simulink model "Main_SpeedOptimisedVersionTannenweg"  (R2024b)
settings: Solver=ode15s  StartTime=0.0  StopTime=3600*2  FixedStep=0.1  RelTol=0.001
model workspace (MAT data in the model file):
  Ti = 5
  fa = 0.00071
  fd = 0.03
  ips = 36
  ma = 0.0013
  md = 0.04
  roomarea1 = 20
  s = 15
libraries: fl_lib x1434, nesl_utility x105, SimscapeFluids_lib x35
(part 7 of 22)

== system Main_SpeedOptimisedVersionTannenweg/OG1/Pipe to 11 ==
  Perfect Insulator3 : fl_lib/Thermal/Thermal Elements/Perfect Insulator  T_specify=off  T_priority=None  T=293.15 K  T_nominal_specify=off  T_nominal_value=1  T_nominal_unit=K
  Pipe (TL)3 : fl_lib/Thermal Liquid/Elements/Pipe (TL)  length=5.32 m  area=fa m^2  Dh=fd m  length_add=1 m  roughness=15e-6 m  Re_lam=2000  Re_tur=4000  shape_factor=64  Nu_lam=3.66  dynamic_compressibility=true  inertia=false  p0=0.101325 MPa  T0=293.15 K  mdot0=0 kg/s
  out : PMIOPort  Side=Right
  in : PMIOPort  Port=2  Side=Left
  connections:
  Perfect Insulator3/LConn1 -- Pipe (TL)3/LConn2
  in/RConn1 -- Pipe (TL)3/LConn1
  out/RConn1 -- Pipe (TL)3/RConn1

== system Main_SpeedOptimisedVersionTannenweg/OG1/Pipe to 12 ==
  Perfect Insulator3 : fl_lib/Thermal/Thermal Elements/Perfect Insulator  T_specify=off  T_priority=None  T=293.15 K  T_nominal_specify=off  T_nominal_value=1  T_nominal_unit=K
  Pipe (TL)3 : fl_lib/Thermal Liquid/Elements/Pipe (TL)  length=7.7 m  area=fa m^2  Dh=fd m  length_add=1 m  roughness=15e-6 m  Re_lam=2000  Re_tur=4000  shape_factor=64  Nu_lam=3.66  dynamic_compressibility=true  inertia=false  p0=0.101325 MPa  T0=293.15 K  mdot0=0 kg/s
  out : PMIOPort  Side=Right
  in : PMIOPort  Port=2  Side=Left
  connections:
  in/RConn1 -- Pipe (TL)3/LConn1
  Perfect Insulator3/LConn1 -- Pipe (TL)3/LConn2
  out/RConn1 -- Pipe (TL)3/RConn1

== system Main_SpeedOptimisedVersionTannenweg/OG1/Pipe to 2 ==
  Perfect Insulator1 : fl_lib/Thermal/Thermal Elements/Perfect Insulator  T_specify=off  T_priority=None  T=293.15 K  T_nominal_specify=off  T_nominal_value=1  T_nominal_unit=K
  Pipe (TL)1 : fl_lib/Thermal Liquid/Elements/Pipe (TL)  length=2.38 m  area=fa m^2  Dh=fd m  length_add=1 m  roughness=15e-6 m  Re_lam=2000  Re_tur=4000  shape_factor=64  Nu_lam=3.66  dynamic_compressibility=true  inertia=false  p0=0.101325 MPa  T0=293.15 K  mdot0=0 kg/s
  " in" : PMIOPort  Side=Left
  out : PMIOPort  Port=2  Side=Right
  connections:
  " in"/RConn1 -- Pipe (TL)1/LConn1
  Perfect Insulator1/LConn1 -- Pipe (TL)1/LConn2
  out/RConn1 -- Pipe (TL)1/RConn1

== system Main_SpeedOptimisedVersionTannenweg/OG1/Pipe to 4 ==
  Perfect Insulator2 : fl_lib/Thermal/Thermal Elements/Perfect Insulator  T_specify=off  T_priority=None  T=293.15 K  T_nominal_specify=off  T_nominal_value=1  T_nominal_unit=K
  Pipe (TL)2 : fl_lib/Thermal Liquid/Elements/Pipe (TL)  length=7.38 m  area=fa m^2  Dh=fd m  length_add=1 m  roughness=15e-6 m  Re_lam=2000  Re_tur=4000  shape_factor=64  Nu_lam=3.66  dynamic_compressibility=true  inertia=false  p0=0.101325 MPa  T0=293.15 K  mdot0=0 kg/s
  in : PMIOPort  Side=Left
  out : PMIOPort  Port=2  Side=Right
  connections:
  Pipe (TL)2/LConn1 -- in/RConn1
  Perfect Insulator2/LConn1 -- Pipe (TL)2/LConn2
  out/RConn1 -- Pipe (TL)2/RConn1

== system Main_SpeedOptimisedVersionTannenweg/OG1/Pipe to 5 ==
  Perfect Insulator3 : fl_lib/Thermal/Thermal Elements/Perfect Insulator  T_specify=off  T_priority=None  T=293.15 K  T_nominal_specify=off  T_nominal_value=1  T_nominal_unit=K
  Pipe (TL)3 : fl_lib/Thermal Liquid/Elements/Pipe (TL)  length=12.42 m  area=fa m^2  Dh=fd m  length_add=1 m  roughness=15e-6 m  Re_lam=2000  Re_tur=4000  shape_factor=64  Nu_lam=3.66  dynamic_compressibility=true  inertia=false  p0=0.101325 MPa  T0=293.15 K  mdot0=0 kg/s
  out : PMIOPort  Side=Right
  " in" : PMIOPort  Port=2  Side=Left
  connections:
  " in"/RConn1 -- Pipe (TL)3/LConn1
  Perfect Insulator3/LConn1 -- Pipe (TL)3/LConn2
  out/RConn1 -- Pipe (TL)3/RConn1

== system Main_SpeedOptimisedVersionTannenweg/OG1/Pipe to 6 ==
  Perfect Insulator3 : fl_lib/Thermal/Thermal Elements/Perfect Insulator  T_specify=off  T_priority=None  T=293.15 K  T_nominal_specify=off  T_nominal_value=1  T_nominal_unit=K
  Pipe (TL)3 : fl_lib/Thermal Liquid/Elements/Pipe (TL)  length=9.34 m  area=fa m^2  Dh=fd m  length_add=1 m  roughness=15e-6 m  Re_lam=2000  Re_tur=4000  shape_factor=64  Nu_lam=3.66  dynamic_compressibility=true  inertia=false  p0=0.101325 MPa  T0=293.15 K  mdot0=0 kg/s
  out : PMIOPort  Side=Right
  " in" : PMIOPort  Port=2  Side=Left
  connections:
  Perfect Insulator3/LConn1 -- Pipe (TL)3/LConn2
  " in"/RConn1 -- Pipe (TL)3/LConn1
  out/RConn1 -- Pipe (TL)3/RConn1

== system Main_SpeedOptimisedVersionTannenweg/OG1/Pipe to 7 ==
  Perfect Insulator3 : fl_lib/Thermal/Thermal Elements/Perfect Insulator  T_specify=off  T_priority=None  T=293.15 K  T_nominal_specify=off  T_nominal_value=1  T_nominal_unit=K
  Pipe (TL)3 : fl_lib/Thermal Liquid/Elements/Pipe (TL)  length=3.5 m  area=fa m^2  Dh=fd m  length_add=1 m  roughness=15e-6 m  Re_lam=2000  Re_tur=4000  shape_factor=64  Nu_lam=3.66  dynamic_compressibility=true  inertia=false  p0=0.101325 MPa  T0=293.15 K  mdot0=0 kg/s
  out : PMIOPort  Side=Right
  " in" : PMIOPort  Port=2  Side=Left
  connections:
  " in"/RConn1 -- Pipe (TL)3/LConn1
  Perfect Insulator3/LConn1 -- Pipe (TL)3/LConn2
  out/RConn1 -- Pipe (TL)3/RConn1

== system Main_SpeedOptimisedVersionTannenweg/OG1/Pipe to 8 ==
  Perfect Insulator3 : fl_lib/Thermal/Thermal Elements/Perfect Insulator  T_specify=off  T_priority=None  T=293.15 K  T_nominal_specify=off  T_nominal_value=1  T_nominal_unit=K
  Pipe (TL)3 : fl_lib/Thermal Liquid/Elements/Pipe (TL)  length=10.04 m  area=fa m^2  Dh=fd m  length_add=1 m  roughness=15e-6 m  Re_lam=2000  Re_tur=4000  shape_factor=64  Nu_lam=3.66  dynamic_compressibility=true  inertia=false  p0=0.101325 MPa  T0=293.15 K  mdot0=0 kg/s
  out : PMIOPort  Side=Right
  in : PMIOPort  Port=2  Side=Left
  connections:
  in/RConn1 -- Pipe (TL)3/LConn1
  Perfect Insulator3/LConn1 -- Pipe (TL)3/LConn2
  out/RConn1 -- Pipe (TL)3/RConn1

== system Main_SpeedOptimisedVersionTannenweg/OG1/Pipe to 9a ==
  Perfect Insulator3 : fl_lib/Thermal/Thermal Elements/Perfect Insulator  T_specify=off  T_priority=None  T=293.15 K  T_nominal_specify=off  T_nominal_value=1  T_nominal_unit=K
  Pipe (TL)3 : fl_lib/Thermal Liquid/Elements/Pipe (TL)  length=10.14 m  area=fa m^2  Dh=fd m  length_add=1 m  roughness=15e-6 m  Re_lam=2000  Re_tur=4000  shape_factor=64  Nu_lam=3.66  dynamic_compressibility=true  inertia=false  p0=0.101325 MPa  T0=293.15 K  mdot0=0 kg/s
  out : PMIOPort  Side=Right
  in : PMIOPort  Port=2  Side=Left
  connections:
  Perfect Insulator3/LConn1 -- Pipe (TL)3/LConn2
  in/RConn1 -- Pipe (TL)3/LConn1
  Pipe (TL)3/RConn1 -- out/RConn1

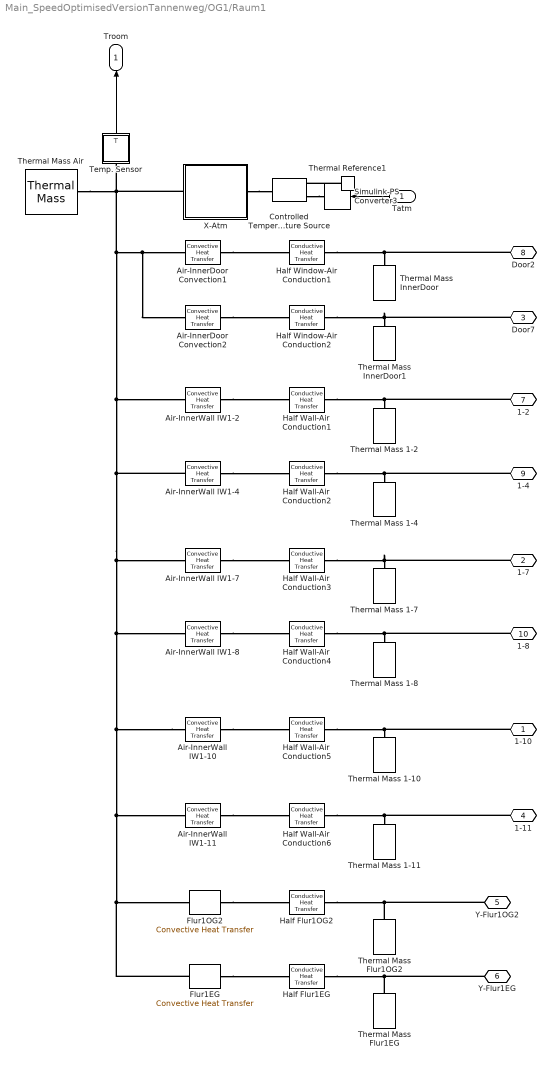
== system Main_SpeedOptimisedVersionTannenweg/OG1/Raum1 ==
  Tatm : Inport
  Air-InnerDoor Convection1 : fl_lib/Thermal/Thermal Elements/Convective Heat Transfer  thermal_type=foundation.enum.constant_variable.constant  area=2 m^2  heat_tr_coeff=.8 W/m^2/K  min_heat_tr_coeff=1e-3 W/(K*m^2)  T_specify=off  T_priority=High  T=0 K  T_nominal_specify=off  T_nominal_value=1  T_nominal_unit=K  Q_specify=off  Q_priority=High  Q=0 J/s  Q_nominal_specify=off  Q_nominal_value=1  Q_nominal_unit=W
  Air-InnerDoor Convection2 : fl_lib/Thermal/Thermal Elements/Convective Heat Transfer  thermal_type=foundation.enum.constant_variable.constant  area=2 m^2  heat_tr_coeff=.8 W/m^2/K  min_heat_tr_coeff=1e-3 W/(K*m^2)  T_specify=off  T_priority=High  T=0 K  T_nominal_specify=off  T_nominal_value=1  T_nominal_unit=K  Q_specify=off  Q_priority=High  Q=0 J/s  Q_nominal_specify=off  Q_nominal_value=1  Q_nominal_unit=W
  Air-InnerWall IW1-10 : fl_lib/Thermal/Thermal Elements/Convective Heat Transfer  thermal_type=foundation.enum.constant_variable.constant  area=3.5 m^2  heat_tr_coeff=.8 W/m^2/K  min_heat_tr_coeff=1e-3 W/(K*m^2)  T_specify=off  T_priority=High  T=0 K  T_nominal_specify=off  T_nominal_value=1  T_nominal_unit=K  Q_specify=off  Q_priority=High  Q=0 J/s  Q_nominal_specify=off  Q_nominal_value=1  Q_nominal_unit=W
  Air-InnerWall IW1-11 : fl_lib/Thermal/Thermal Elements/Convective Heat Transfer  thermal_type=foundation.enum.constant_variable.constant  area=3.7 m^2  heat_tr_coeff=.8 W/m^2/K  min_heat_tr_coeff=1e-3 W/(K*m^2)  T_specify=off  T_priority=High  T=0 K  T_nominal_specify=off  T_nominal_value=1  T_nominal_unit=K  Q_specify=off  Q_priority=High  Q=0 J/s  Q_nominal_specify=off  Q_nominal_value=1  Q_nominal_unit=W
  Air-InnerWall IW1-2 : fl_lib/Thermal/Thermal Elements/Convective Heat Transfer  thermal_type=foundation.enum.constant_variable.constant  area=3.8 m^2  heat_tr_coeff=.8 W/m^2/K  min_heat_tr_coeff=1e-3 W/(K*m^2)  T_specify=off  T_priority=High  T=0 K  T_nominal_specify=off  T_nominal_value=1  T_nominal_unit=K  Q_specify=off  Q_priority=High  Q=0 J/s  Q_nominal_specify=off  Q_nominal_value=1  Q_nominal_unit=W
  Air-InnerWall IW1-4 : fl_lib/Thermal/Thermal Elements/Convective Heat Transfer  thermal_type=foundation.enum.constant_variable.constant  area=7.2 m^2  heat_tr_coeff=.8 W/m^2/K  min_heat_tr_coeff=1e-3 W/(K*m^2)  T_specify=off  T_priority=High  T=0 K  T_nominal_specify=off  T_nominal_value=1  T_nominal_unit=K  Q_specify=off  Q_priority=High  Q=0 J/s  Q_nominal_specify=off  Q_nominal_value=1  Q_nominal_unit=W
  Air-InnerWall IW1-7 : fl_lib/Thermal/Thermal Elements/Convective Heat Transfer  thermal_type=foundation.enum.constant_variable.constant  area=3.1 m^2  heat_tr_coeff=.8 W/m^2/K  min_heat_tr_coeff=1e-3 W/(K*m^2)  T_specify=off  T_priority=High  T=0 K  T_nominal_specify=off  T_nominal_value=1  T_nominal_unit=K  Q_specify=off  Q_priority=High  Q=0 J/s  Q_nominal_specify=off  Q_nominal_value=1  Q_nominal_unit=W
  Air-InnerWall IW1-8 : fl_lib/Thermal/Thermal Elements/Convective Heat Transfer  thermal_type=foundation.enum.constant_variable.constant  area=7.9 m^2  heat_tr_coeff=.8 W/m^2/K  min_heat_tr_coeff=1e-3 W/(K*m^2)  T_specify=off  T_priority=High  T=0 K  T_nominal_specify=off  T_nominal_value=1  T_nominal_unit=K  Q_specify=off  Q_priority=High  Q=0 J/s  Q_nominal_specify=off  Q_nominal_value=1  Q_nominal_unit=W
  Controlled Temperature Source : fl_lib/Thermal/Thermal Sources/Controlled Temperature Source
  Flur1EG : fl_lib/Thermal/Thermal Elements/Convective Heat Transfer  thermal_type=foundation.enum.constant_variable.constant  area=10.76 m^2  heat_tr_coeff=.8 W/m^2/K  min_heat_tr_coeff=1e-3 W/(K*m^2)  T_specify=off  T_priority=High  T=0 K  T_nominal_specify=off  T_nominal_value=1  T_nominal_unit=K  Q_specify=off  Q_priority=High  Q=0 J/s  Q_nominal_specify=off  Q_nominal_value=1  Q_nominal_unit=W
  Flur1OG2 : fl_lib/Thermal/Thermal Elements/Convective Heat Transfer  thermal_type=foundation.enum.constant_variable.constant  area=10.76 m^2  heat_tr_coeff=.8 W/m^2/K  min_heat_tr_coeff=1e-3 W/(K*m^2)  T_specify=off  T_priority=High  T=0 K  T_nominal_specify=off  T_nominal_value=1  T_nominal_unit=K  Q_specify=off  Q_priority=High  Q=0 J/s  Q_nominal_specify=off  Q_nominal_value=1  Q_nominal_unit=W
  Half Flur1EG : fl_lib/Thermal/Thermal Elements/Conductive Heat Transfer  thermal_type=foundation.enum.ConstantVariableTabulated.Constant  wall_geometry=foundation.enum.ConductionWallGeometry.Planar  area=10.76 m^2  thickness=.15 m  d_in=0.05 m  d_out=0.1 m  L=1 m  th_cond_min=10 W/(K*m)  th_cond=.32 W/m/K  th_cond_TLU=[413, 401, 392, 383, 371, 357, 342] W/(K*m)  temp_TLU=[200, 273, 400, 600, 800, 1000, 1200] K  T_specify=off  T_priority=High  T=0 K  T_nominal_specify=off  T_nominal_value=1  T_nominal_unit=K  Q_specify=off  Q_priority=High  Q=0 J/s  Q_nominal_specify=off  Q_nominal_value=1  Q_nominal_unit=W
  Half Flur1OG2 : fl_lib/Thermal/Thermal Elements/Conductive Heat Transfer  thermal_type=foundation.enum.ConstantVariableTabulated.Constant  wall_geometry=foundation.enum.ConductionWallGeometry.Planar  area=10.76 m^2  thickness=.15 m  d_in=0.05 m  d_out=0.1 m  L=1 m  th_cond_min=10 W/(K*m)  th_cond=.32 W/m/K  th_cond_TLU=[413, 401, 392, 383, 371, 357, 342] W/(K*m)  temp_TLU=[200, 273, 400, 600, 800, 1000, 1200] K  T_specify=off  T_priority=High  T=0 K  T_nominal_specify=off  T_nominal_value=1  T_nominal_unit=K  Q_specify=off  Q_priority=High  Q=0 J/s  Q_nominal_specify=off  Q_nominal_value=1  Q_nominal_unit=W
  Half Wall-Air Conduction1 : fl_lib/Thermal/Thermal Elements/Conductive Heat Transfer  thermal_type=foundation.enum.ConstantVariableTabulated.Constant  wall_geometry=foundation.enum.ConductionWallGeometry.Planar  area=3.8 m^2  thickness=.16 m  d_in=0.05 m  d_out=0.1 m  L=1 m  th_cond_min=10 W/(K*m)  th_cond=.069 W/m/K  th_cond_TLU=[413, 401, 392, 383, 371, 357, 342] W/(K*m)  temp_TLU=[200, 273, 400, 600, 800, 1000, 1200] K  T_specify=off  T_priority=High  T=0 K  T_nominal_specify=off  T_nominal_value=1  T_nominal_unit=K  Q_specify=off  Q_priority=High  Q=0 J/s  Q_nominal_specify=off  Q_nominal_value=1  Q_nominal_unit=W
  Half Wall-Air Conduction2 : fl_lib/Thermal/Thermal Elements/Conductive Heat Transfer  thermal_type=foundation.enum.ConstantVariableTabulated.Constant  wall_geometry=foundation.enum.ConductionWallGeometry.Planar  area=7.2 m^2  thickness=.16 m  d_in=0.05 m  d_out=0.1 m  L=1 m  th_cond_min=10 W/(K*m)  th_cond=.069 W/m/K  th_cond_TLU=[413, 401, 392, 383, 371, 357, 342] W/(K*m)  temp_TLU=[200, 273, 400, 600, 800, 1000, 1200] K  T_specify=off  T_priority=High  T=0 K  T_nominal_specify=off  T_nominal_value=1  T_nominal_unit=K  Q_specify=off  Q_priority=High  Q=0 J/s  Q_nominal_specify=off  Q_nominal_value=1  Q_nominal_unit=W
  Half Wall-Air Conduction3 : fl_lib/Thermal/Thermal Elements/Conductive Heat Transfer  thermal_type=foundation.enum.ConstantVariableTabulated.Constant  wall_geometry=foundation.enum.ConductionWallGeometry.Planar  area=3.1 m^2  thickness=.16 m  d_in=0.05 m  d_out=0.1 m  L=1 m  th_cond_min=10 W/(K*m)  th_cond=.069 W/m/K  th_cond_TLU=[413, 401, 392, 383, 371, 357, 342] W/(K*m)  temp_TLU=[200, 273, 400, 600, 800, 1000, 1200] K  T_specify=off  T_priority=High  T=0 K  T_nominal_specify=off  T_nominal_value=1  T_nominal_unit=K  Q_specify=off  Q_priority=High  Q=0 J/s  Q_nominal_specify=off  Q_nominal_value=1  Q_nominal_unit=W
  Half Wall-Air Conduction4 : fl_lib/Thermal/Thermal Elements/Conductive Heat Transfer  thermal_type=foundation.enum.ConstantVariableTabulated.Constant  wall_geometry=foundation.enum.ConductionWallGeometry.Planar  area=7.9 m^2  thickness=.16 m  d_in=0.05 m  d_out=0.1 m  L=1 m  th_cond_min=10 W/(K*m)  th_cond=.069 W/m/K  th_cond_TLU=[413, 401, 392, 383, 371, 357, 342] W/(K*m)  temp_TLU=[200, 273, 400, 600, 800, 1000, 1200] K  T_specify=off  T_priority=High  T=0 K  T_nominal_specify=off  T_nominal_value=1  T_nominal_unit=K  Q_specify=off  Q_priority=High  Q=0 J/s  Q_nominal_specify=off  Q_nominal_value=1  Q_nominal_unit=W
  Half Wall-Air Conduction5 : fl_lib/Thermal/Thermal Elements/Conductive Heat Transfer  thermal_type=foundation.enum.ConstantVariableTabulated.Constant  wall_geometry=foundation.enum.ConductionWallGeometry.Planar  area=3.5 m^2  thickness=.16 m  d_in=0.05 m  d_out=0.1 m  L=1 m  th_cond_min=10 W/(K*m)  th_cond=.069 W/m/K  th_cond_TLU=[413, 401, 392, 383, 371, 357, 342] W/(K*m)  temp_TLU=[200, 273, 400, 600, 800, 1000, 1200] K  T_specify=off  T_priority=High  T=0 K  T_nominal_specify=off  T_nominal_value=1  T_nominal_unit=K  Q_specify=off  Q_priority=High  Q=0 J/s  Q_nominal_specify=off  Q_nominal_value=1  Q_nominal_unit=W
  Half Wall-Air Conduction6 : fl_lib/Thermal/Thermal Elements/Conductive Heat Transfer  thermal_type=foundation.enum.ConstantVariableTabulated.Constant  wall_geometry=foundation.enum.ConductionWallGeometry.Planar  area=3.7 m^2  thickness=.16 m  d_in=0.05 m  d_out=0.1 m  L=1 m  th_cond_min=10 W/(K*m)  th_cond=.069 W/m/K  th_cond_TLU=[413, 401, 392, 383, 371, 357, 342] W/(K*m)  temp_TLU=[200, 273, 400, 600, 800, 1000, 1200] K  T_specify=off  T_priority=High  T=0 K  T_nominal_specify=off  T_nominal_value=1  T_nominal_unit=K  Q_specify=off  Q_priority=High  Q=0 J/s  Q_nominal_specify=off  Q_nominal_value=1  Q_nominal_unit=W
  Half Window-Air Conduction1 : fl_lib/Thermal/Thermal Elements/Conductive Heat Transfer  thermal_type=foundation.enum.ConstantVariableTabulated.Constant  wall_geometry=foundation.enum.ConductionWallGeometry.Planar  area=2 m^2  thickness=.022 m  d_in=0.05 m  d_out=0.1 m  L=1 m  th_cond_min=10 W/(K*m)  th_cond=.13 W/m/K  th_cond_TLU=[413, 401, 392, 383, 371, 357, 342] W/(K*m)  temp_TLU=[200, 273, 400, 600, 800, 1000, 1200] K  T_specify=off  T_priority=High  T=0 K  T_nominal_specify=off  T_nominal_value=1  T_nominal_unit=K  Q_specify=off  Q_priority=High  Q=0 J/s  Q_nominal_specify=off  Q_nominal_value=1  Q_nominal_unit=W
  Half Window-Air Conduction2 : fl_lib/Thermal/Thermal Elements/Conductive Heat Transfer  thermal_type=foundation.enum.ConstantVariableTabulated.Constant  wall_geometry=foundation.enum.ConductionWallGeometry.Planar  area=2 m^2  thickness=.022 m  d_in=0.05 m  d_out=0.1 m  L=1 m  th_cond_min=10 W/(K*m)  th_cond=.13 W/m/K  th_cond_TLU=[413, 401, 392, 383, 371, 357, 342] W/(K*m)  temp_TLU=[200, 273, 400, 600, 800, 1000, 1200] K  T_specify=off  T_priority=High  T=0 K  T_nominal_specify=off  T_nominal_value=1  T_nominal_unit=K  Q_specify=off  Q_priority=High  Q=0 J/s  Q_nominal_specify=off  Q_nominal_value=1  Q_nominal_unit=W
  Simulink-PS Converter3 : nesl_utility/Simulink-PS Converter  PhysicalDomain=network_engine_domain  SubClassName=ps_input  LeftPortType=input  RightPortType=output  PseudoPeriodic=off  Frequencies=[]  NoiseDistribution=none  NoiseParameters=[]  Unit=degC  AffineConversion=on  FilteringAndDerivatives=zero  SimscapeFilterOrder=1  InputFilterTimeConstant=.001  UdotUserProvided=0
  Temp. Sensor : Subsystem
  Thermal Mass 1-10 : fl_lib/Thermal/Thermal Elements/Thermal Mass  mass_type=foundation.enum.constant_variable.constant  mass=3.5*.15*547 kg  sp_heat=876 J/kg/K  mass_min=1e-6 kg  num_ports=foundation.enum.numPorts2.one  m_specify=off  m_priority=High  m=1 kg  m_nominal_specify=off  m_nominal_value=1  m_nominal_unit=kg  T_specify=on  T_priority=High  T=Ti degC  T_nominal_specify=off  T_nominal_value=1  T_nominal_unit=K  Q_specify=off  Q_priority=None  Q=0 W  Q_nominal_specify=off  Q_nominal_value=1  Q_nominal_unit=W
  Thermal Mass 1-11 : fl_lib/Thermal/Thermal Elements/Thermal Mass  mass_type=foundation.enum.constant_variable.constant  mass=3.7*.15*547 kg  sp_heat=876 J/kg/K  mass_min=1e-6 kg  num_ports=foundation.enum.numPorts2.one  m_specify=off  m_priority=High  m=1 kg  m_nominal_specify=off  m_nominal_value=1  m_nominal_unit=kg  T_specify=on  T_priority=High  T=Ti degC  T_nominal_specify=off  T_nominal_value=1  T_nominal_unit=K  Q_specify=off  Q_priority=None  Q=0 W  Q_nominal_specify=off  Q_nominal_value=1  Q_nominal_unit=W
  Thermal Mass 1-2 : fl_lib/Thermal/Thermal Elements/Thermal Mass  mass_type=foundation.enum.constant_variable.constant  mass=3.8*.15*547 kg  sp_heat=876 J/kg/K  mass_min=1e-6 kg  num_ports=foundation.enum.numPorts2.one  m_specify=off  m_priority=High  m=1 kg  m_nominal_specify=off  m_nominal_value=1  m_nominal_unit=kg  T_specify=on  T_priority=High  T=Ti degC  T_nominal_specify=off  T_nominal_value=1  T_nominal_unit=K  Q_specify=off  Q_priority=None  Q=0 W  Q_nominal_specify=off  Q_nominal_value=1  Q_nominal_unit=W
  Thermal Mass 1-4 : fl_lib/Thermal/Thermal Elements/Thermal Mass  mass_type=foundation.enum.constant_variable.constant  mass=7.2*.15*547 kg  sp_heat=876 J/kg/K  mass_min=1e-6 kg  num_ports=foundation.enum.numPorts2.one  m_specify=off  m_priority=High  m=1 kg  m_nominal_specify=off  m_nominal_value=1  m_nominal_unit=kg  T_specify=on  T_priority=High  T=Ti degC  T_nominal_specify=off  T_nominal_value=1  T_nominal_unit=K  Q_specify=off  Q_priority=None  Q=0 W  Q_nominal_specify=off  Q_nominal_value=1  Q_nominal_unit=W
  Thermal Mass 1-7 : fl_lib/Thermal/Thermal Elements/Thermal Mass  mass_type=foundation.enum.constant_variable.constant  mass=3.1*.15*547 kg  sp_heat=876 J/kg/K  mass_min=1e-6 kg  num_ports=foundation.enum.numPorts2.one  m_specify=off  m_priority=High  m=1 kg  m_nominal_specify=off  m_nominal_value=1  m_nominal_unit=kg  T_specify=on  T_priority=High  T=Ti degC  T_nominal_specify=off  T_nominal_value=1  T_nominal_unit=K  Q_specify=off  Q_priority=None  Q=0 W  Q_nominal_specify=off  Q_nominal_value=1  Q_nominal_unit=W
  Thermal Mass 1-8 : fl_lib/Thermal/Thermal Elements/Thermal Mass  mass_type=foundation.enum.constant_variable.constant  mass=7.9*.15*547 kg  sp_heat=876 J/kg/K  mass_min=1e-6 kg  num_ports=foundation.enum.numPorts2.one  m_specify=off  m_priority=High  m=1 kg  m_nominal_specify=off  m_nominal_value=1  m_nominal_unit=kg  T_specify=on  T_priority=High  T=Ti degC  T_nominal_specify=off  T_nominal_value=1  T_nominal_unit=K  Q_specify=off  Q_priority=None  Q=0 W  Q_nominal_specify=off  Q_nominal_value=1  Q_nominal_unit=W
  Thermal Mass Air : fl_lib/Thermal/Thermal Elements/Thermal Mass  mass_type=foundation.enum.constant_variable.constant  mass=13.9 kg  sp_heat=1005 J/kg/K  mass_min=1e-6 kg  num_ports=foundation.enum.numPorts2.one  m_specify=off  m_priority=High  m=1 kg  m_nominal_specify=off  m_nominal_value=1  m_nominal_unit=kg  T_specify=on  T_priority=High  T=Ti degC  T_nominal_specify=off  T_nominal_value=1  T_nominal_unit=K  Q_specify=off  Q_priority=None  Q=0 W  Q_nominal_specify=off  Q_nominal_value=1  Q_nominal_unit=W
  Thermal Mass Flur1EG : fl_lib/Thermal/Thermal Elements/Thermal Mass  mass_type=foundation.enum.constant_variable.constant  mass=3033 kg  sp_heat=889 J/kg/K  mass_min=1e-6 kg  num_ports=foundation.enum.numPorts2.one  m_specify=off  m_priority=High  m=1 kg  m_nominal_specify=off  m_nominal_value=1  m_nominal_unit=kg  T_specify=on  T_priority=High  T=Ti degC  T_nominal_specify=off  T_nominal_value=1  T_nominal_unit=K  Q_specify=off  Q_priority=None  Q=0 W  Q_nominal_specify=off  Q_nominal_value=1  Q_nominal_unit=W
  Thermal Mass Flur1OG2 : fl_lib/Thermal/Thermal Elements/Thermal Mass  mass_type=foundation.enum.constant_variable.constant  mass=3033 kg  sp_heat=889 J/kg/K  mass_min=1e-6 kg  num_ports=foundation.enum.numPorts2.one  m_specify=off  m_priority=High  m=1 kg  m_nominal_specify=off  m_nominal_value=1  m_nominal_unit=kg  T_specify=on  T_priority=High  T=Ti degC  T_nominal_specify=off  T_nominal_value=1  T_nominal_unit=K  Q_specify=off  Q_priority=None  Q=0 W  Q_nominal_specify=off  Q_nominal_value=1  Q_nominal_unit=W
  Thermal Mass InnerDoor : fl_lib/Thermal/Thermal Elements/Thermal Mass  mass_type=foundation.enum.constant_variable.constant  mass=2*.022*450 kg  sp_heat=1600 J/kg/K  mass_min=1e-6 kg  num_ports=foundation.enum.numPorts2.one  m_specify=off  m_priority=High  m=1 kg  m_nominal_specify=off  m_nominal_value=1  m_nominal_unit=kg  T_specify=on  T_priority=High  T=Ti degC  T_nominal_specify=off  T_nominal_value=1  T_nominal_unit=K  Q_specify=off  Q_priority=None  Q=0 W  Q_nominal_specify=off  Q_nominal_value=1  Q_nominal_unit=W
  Thermal Mass InnerDoor1 : fl_lib/Thermal/Thermal Elements/Thermal Mass  mass_type=foundation.enum.constant_variable.constant  mass=2*.022*450 kg  sp_heat=1600 J/kg/K  mass_min=1e-6 kg  num_ports=foundation.enum.numPorts2.one  m_specify=off  m_priority=High  m=1 kg  m_nominal_specify=off  m_nominal_value=1  m_nominal_unit=kg  T_specify=on  T_priority=High  T=Ti degC  T_nominal_specify=off  T_nominal_value=1  T_nominal_unit=K  Q_specify=off  Q_priority=None  Q=0 W  Q_nominal_specify=off  Q_nominal_value=1  Q_nominal_unit=W
  Thermal Reference1 : fl_lib/Thermal/Thermal Elements/Thermal Reference
  X-Atm : Subsystem
  1-10 : PMIOPort  Side=Left
  1-7 : PMIOPort  Port=2  Side=Left
  Door7 : PMIOPort  Port=3  Side=Left
  1-11 : PMIOPort  Port=4  Side=Left
  Y-Flur1OG2 : PMIOPort  Port=5  Side=Left
  Y-Flur1EG : PMIOPort  Port=6  Side=Left
  1-2 : PMIOPort  Port=7  Side=Right
  Door2 : PMIOPort  Port=8  Side=Right
  1-4 : PMIOPort  Port=9  Side=Right
  1-8 : PMIOPort  Port=10  Side=Right
  Troom : Outport
  wires:
  Temp. Sensor/1(T) -> Troom/1
  Tatm/1 -> Simulink-PS Converter3/1
  connections:
  Flur1OG2/RConn1 -- Half Flur1OG2/LConn1
  Half Flur1OG2/RConn1 -- Y-Flur1OG2/RConn1 -- Thermal Mass Flur1OG2/LConn1
  Air-InnerDoor Convection1/RConn1 -- Half Window-Air Conduction1/LConn1
  Air-InnerWall IW1-11/RConn1 -- Half Wall-Air Conduction6/LConn1
  Air-InnerWall IW1-7/RConn1 -- Half Wall-Air Conduction3/LConn1
  Air-InnerWall IW1-10/RConn1 -- Half Wall-Air Conduction5/LConn1
  Air-InnerDoor Convection2/RConn1 -- Half Window-Air Conduction2/LConn1
  Air-InnerWall IW1-2/RConn1 -- Half Wall-Air Conduction1/LConn1
  Air-InnerWall IW1-4/RConn1 -- Half Wall-Air Conduction2/LConn1
  Air-InnerWall IW1-8/RConn1 -- Half Wall-Air Conduction4/LConn1
  1-10/RConn1 -- Thermal Mass 1-10/LConn1 -- Half Wall-Air Conduction5/RConn1
  Thermal Mass 1-7/LConn1 -- Half Wall-Air Conduction3/RConn1 -- 1-7/RConn1
  Half Wall-Air Conduction6/RConn1 -- Thermal Mass 1-11/LConn1 -- 1-11/RConn1
  Door2/RConn1 -- Thermal Mass InnerDoor/LConn1 -- Half Window-Air Conduction1/RConn1
  Thermal Mass InnerDoor1/LConn1 -- Door7/RConn1 -- Half Window-Air Conduction2/RConn1
  Half Wall-Air Conduction2/RConn1 -- Thermal Mass 1-4/LConn1 -- 1-4/RConn1
  Half Wall-Air Conduction4/RConn1 -- Thermal Mass 1-8/LConn1 -- 1-8/RConn1
  1-2/RConn1 -- Thermal Mass 1-2/LConn1 -- Half Wall-Air Conduction1/RConn1
  Thermal Reference1/LConn1 -- Controlled Temperature Source/RConn2
  Controlled Temperature Source/RConn1 -- Simulink-PS Converter3/RConn1
  Air-InnerWall IW1-10/LConn1 -- Flur1EG/LConn1 -- Flur1OG2/LConn1 -- Air-InnerWall IW1-11/LConn1 -- Thermal Mass Air/LConn1 -- Temp. Sensor/LConn1 -- X-Atm/LConn1 -- Air-InnerDoor Convection1/LConn1 -- Air-InnerDoor Convection2/LConn1 -- Air-InnerWall IW1-2/LConn1 -- Air-InnerWall IW1-4/LConn1 -- Air-InnerWall IW1-7/LConn1 -- Air-InnerWall IW1-8/LConn1
  X-Atm/RConn1 -- Controlled Temperature Source/LConn1
  Half Flur1EG/RConn1 -- Thermal Mass Flur1EG/LConn1 -- Y-Flur1EG/RConn1
  Flur1EG/RConn1 -- Half Flur1EG/LConn1

== system Main_SpeedOptimisedVersionTannenweg/OG1/Raum10 ==
  valve command : Inport
  Tatm : Inport  Port=2
  Air-InnerDoor Convection1 : fl_lib/Thermal/Thermal Elements/Convective Heat Transfer  thermal_type=foundation.enum.constant_variable.constant  area=1.8 m^2  heat_tr_coeff=.8 W/m^2/K  min_heat_tr_coeff=1e-3 W/(K*m^2)  T_specify=off  T_priority=High  T=0 K  T_nominal_specify=off  T_nominal_value=1  T_nominal_unit=K  Q_specify=off  Q_priority=High  Q=0 J/s  Q_nominal_specify=off  Q_nominal_value=1  Q_nominal_unit=W
  Controlled Temperature Source : fl_lib/Thermal/Thermal Sources/Controlled Temperature Source
  Flur10EG : fl_lib/Thermal/Thermal Elements/Convective Heat Transfer  thermal_type=foundation.enum.constant_variable.constant  area=14.51 m^2  heat_tr_coeff=.8 W/m^2/K  min_heat_tr_coeff=1e-3 W/(K*m^2)  T_specify=off  T_priority=High  T=0 K  T_nominal_specify=off  T_nominal_value=1  T_nominal_unit=K  Q_specify=off  Q_priority=High  Q=0 J/s  Q_nominal_specify=off  Q_nominal_value=1  Q_nominal_unit=W
  Flur10OG2 : fl_lib/Thermal/Thermal Elements/Convective Heat Transfer  thermal_type=foundation.enum.constant_variable.constant  area=14.51 m^2  heat_tr_coeff=.8 W/m^2/K  min_heat_tr_coeff=1e-3 W/(K*m^2)  T_specify=off  T_priority=High  T=0 K  T_nominal_specify=off  T_nominal_value=1  T_nominal_unit=K  Q_specify=off  Q_priority=High  Q=0 J/s  Q_nominal_specify=off  Q_nominal_value=1  Q_nominal_unit=W
  Half Flur10EG : fl_lib/Thermal/Thermal Elements/Conductive Heat Transfer  thermal_type=foundation.enum.ConstantVariableTabulated.Constant  wall_geometry=foundation.enum.ConductionWallGeometry.Planar  area=14.51 m^2  thickness=.15 m  d_in=0.05 m  d_out=0.1 m  L=1 m  th_cond_min=10 W/(K*m)  th_cond=.32 W/m/K  th_cond_TLU=[413, 401, 392, 383, 371, 357, 342] W/(K*m)  temp_TLU=[200, 273, 400, 600, 800, 1000, 1200] K  T_specify=off  T_priority=High  T=0 K  T_nominal_specify=off  T_nominal_value=1  T_nominal_unit=K  Q_specify=off  Q_priority=High  Q=0 J/s  Q_nominal_specify=off  Q_nominal_value=1  Q_nominal_unit=W
  Half Flur10OG2 : fl_lib/Thermal/Thermal Elements/Conductive Heat Transfer  thermal_type=foundation.enum.ConstantVariableTabulated.Constant  wall_geometry=foundation.enum.ConductionWallGeometry.Planar  area=14.51 m^2  thickness=.15 m  d_in=0.05 m  d_out=0.1 m  L=1 m  th_cond_min=10 W/(K*m)  th_cond=.32 W/m/K  th_cond_TLU=[413, 401, 392, 383, 371, 357, 342] W/(K*m)  temp_TLU=[200, 273, 400, 600, 800, 1000, 1200] K  T_specify=off  T_priority=High  T=0 K  T_nominal_specify=off  T_nominal_value=1  T_nominal_unit=K  Q_specify=off  Q_priority=High  Q=0 J/s  Q_nominal_specify=off  Q_nominal_value=1  Q_nominal_unit=W
  Half Wall-Air Conduction1 : fl_lib/Thermal/Thermal Elements/Conductive Heat Transfer  thermal_type=foundation.enum.ConstantVariableTabulated.Constant  wall_geometry=foundation.enum.ConductionWallGeometry.Planar  area=3.7 m^2  thickness=.16 m  d_in=0.05 m  d_out=0.1 m  L=1 m  th_cond_min=10 W/(K*m)  th_cond=.069 W/m/K  th_cond_TLU=[413, 401, 392, 383, 371, 357, 342] W/(K*m)  temp_TLU=[200, 273, 400, 600, 800, 1000, 1200] K  T_specify=off  T_priority=High  T=0 K  T_nominal_specify=off  T_nominal_value=1  T_nominal_unit=K  Q_specify=off  Q_priority=High  Q=0 J/s  Q_nominal_specify=off  Q_nominal_value=1  Q_nominal_unit=W
  Half Wall-Air Conduction2 : fl_lib/Thermal/Thermal Elements/Conductive Heat Transfer  thermal_type=foundation.enum.ConstantVariableTabulated.Constant  wall_geometry=foundation.enum.ConductionWallGeometry.Planar  area=1.8 m^2  thickness=.16 m  d_in=0.05 m  d_out=0.1 m  L=1 m  th_cond_min=10 W/(K*m)  th_cond=.069 W/m/K  th_cond_TLU=[413, 401, 392, 383, 371, 357, 342] W/(K*m)  temp_TLU=[200, 273, 400, 600, 800, 1000, 1200] K  T_specify=off  T_priority=High  T=0 K  T_nominal_specify=off  T_nominal_value=1  T_nominal_unit=K  Q_specify=off  Q_priority=High  Q=0 J/s  Q_nominal_specify=off  Q_nominal_value=1  Q_nominal_unit=W
  Half Wall-Air Conduction3 : fl_lib/Thermal/Thermal Elements/Conductive Heat Transfer  thermal_type=foundation.enum.ConstantVariableTabulated.Constant  wall_geometry=foundation.enum.ConductionWallGeometry.Planar  area=12.5 m^2  thickness=.16 m  d_in=0.05 m  d_out=0.1 m  L=1 m  th_cond_min=10 W/(K*m)  th_cond=.069 W/m/K  th_cond_TLU=[413, 401, 392, 383, 371, 357, 342] W/(K*m)  temp_TLU=[200, 273, 400, 600, 800, 1000, 1200] K  T_specify=off  T_priority=High  T=0 K  T_nominal_specify=off  T_nominal_value=1  T_nominal_unit=K  Q_specify=off  Q_priority=High  Q=0 J/s  Q_nominal_specify=off  Q_nominal_value=1  Q_nominal_unit=W
  Half Wall-Air Conduction4 : fl_lib/Thermal/Thermal Elements/Conductive Heat Transfer  thermal_type=foundation.enum.ConstantVariableTabulated.Constant  wall_geometry=foundation.enum.ConductionWallGeometry.Planar  area=12.5 m^2  thickness=.16 m  d_in=0.05 m  d_out=0.1 m  L=1 m  th_cond_min=10 W/(K*m)  th_cond=.069 W/m/K  th_cond_TLU=[413, 401, 392, 383, 371, 357, 342] W/(K*m)  temp_TLU=[200, 273, 400, 600, 800, 1000, 1200] K  T_specify=off  T_priority=High  T=0 K  T_nominal_specify=off  T_nominal_value=1  T_nominal_unit=K  Q_specify=off  Q_priority=High  Q=0 J/s  Q_nominal_specify=off  Q_nominal_value=1  Q_nominal_unit=W
  Half Window-Air Conduction1 : fl_lib/Thermal/Thermal Elements/Conductive Heat Transfer  thermal_type=foundation.enum.ConstantVariableTabulated.Constant  wall_geometry=foundation.enum.ConductionWallGeometry.Planar  area=1.8 m^2  thickness=.022 m  d_in=0.05 m  d_out=0.1 m  L=1 m  th_cond_min=10 W/(K*m)  th_cond=.13 W/m/K  th_cond_TLU=[413, 401, 392, 383, 371, 357, 342] W/(K*m)  temp_TLU=[200, 273, 400, 600, 800, 1000, 1200] K  T_specify=off  T_priority=High  T=0 K  T_nominal_specify=off  T_nominal_value=1  T_nominal_unit=K  Q_specify=off  Q_priority=High  Q=0 J/s  Q_nominal_specify=off  Q_nominal_value=1  Q_nominal_unit=W
  Heater : Subsystem
      settings: PortSchema="{\"entries\":[{\"content\":{\"sides\":[{\"content\":{\"connectorIds\":[\"In1\"]},\"type\":\"ConnectorPlacement.EquallySpacedRectSide\",\"uuid\":\"7b4379d5-fe86-4f5f-b347-17463247d5cb\"},{\"content\":{\"connectorIds\":[\"RConn1\"],\"side\":\"RIGHT\"},\"type\":\"ConnectorPlacement.EquallySpacedRectSide\",\"uuid\":\"add3919f-9a79-4726-aacf-5344366c736f\"},{\"content\":{\"connectorIds\":[\"LConn1\"],\"side\":\"TOP\"},\"type\":\"ConnectorPlacement.EquallySpacedRectSide\",\"uuid\":\"2be7b118-9114-410d-904a-4756a3068fbb\"},{\"content\":{\"connectorIds\":[\"RConn2\"],\"side\":\"BOTTOM\"},\"type\":\"ConnectorPlacement.EquallySpacedRectSide\",\"uuid\":\"3477f1e1-5c09-4719-a7a1-17d4fd79a7ad\"}]},\"type\":\"ConnectorPlacement.EquallySpacedConnector\",\"uuid\":\"01d92670-8519-469a-8463-0c3952b88216\"}],\"packageUris\":[\"http://schema.mathworks.com/mf0/Connector/R2020b\"],\"version\":\"1.0\"}"
  IW10-1 : fl_lib/Thermal/Thermal Elements/Convective Heat Transfer  thermal_type=foundation.enum.constant_variable.constant  area=1 m^2  heat_tr_coeff=.8 W/m^2/K  min_heat_tr_coeff=1e-3 W/(K*m^2)  T_specify=off  T_priority=High  T=0 K  T_nominal_specify=off  T_nominal_value=1  T_nominal_unit=K  Q_specify=off  Q_priority=High  Q=0 J/s  Q_nominal_specify=off  Q_nominal_value=1  Q_nominal_unit=W
  IW10-11 : fl_lib/Thermal/Thermal Elements/Convective Heat Transfer  thermal_type=foundation.enum.constant_variable.constant  area=12.5 m^2  heat_tr_coeff=.8 W/m^2/K  min_heat_tr_coeff=1e-3 W/(K*m^2)  T_specify=off  T_priority=High  T=0 K  T_nominal_specify=off  T_nominal_value=1  T_nominal_unit=K  Q_specify=off  Q_priority=High  Q=0 J/s  Q_nominal_specify=off  Q_nominal_value=1  Q_nominal_unit=W
  IW10-7 : fl_lib/Thermal/Thermal Elements/Convective Heat Transfer  thermal_type=foundation.enum.constant_variable.constant  area=1.8 m^2  heat_tr_coeff=.8 W/m^2/K  min_heat_tr_coeff=1e-3 W/(K*m^2)  T_specify=off  T_priority=High  T=0 K  T_nominal_specify=off  T_nominal_value=1  T_nominal_unit=K  Q_specify=off  Q_priority=High  Q=0 J/s  Q_nominal_specify=off  Q_nominal_value=1  Q_nominal_unit=W
  IW10-9 : fl_lib/Thermal/Thermal Elements/Convective Heat Transfer  thermal_type=foundation.enum.constant_variable.constant  area=12.5 m^2  heat_tr_coeff=.8 W/m^2/K  min_heat_tr_coeff=1e-3 W/(K*m^2)  T_specify=off  T_priority=High  T=0 K  T_nominal_specify=off  T_nominal_value=1  T_nominal_unit=K  Q_specify=off  Q_priority=High  Q=0 J/s  Q_nominal_specify=off  Q_nominal_value=1  Q_nominal_unit=W
  Simulink-PS Converter3 : nesl_utility/Simulink-PS Converter  PhysicalDomain=network_engine_domain  SubClassName=ps_input  LeftPortType=input  RightPortType=output  PseudoPeriodic=off  Frequencies=[]  NoiseDistribution=none  NoiseParameters=[]  Unit=degC  AffineConversion=on  FilteringAndDerivatives=zero  SimscapeFilterOrder=1  InputFilterTimeConstant=.001  UdotUserProvided=0
  Temp. Sensor : Subsystem
  Thermal Mass 10-1 : fl_lib/Thermal/Thermal Elements/Thermal Mass  mass_type=foundation.enum.constant_variable.constant  mass=547*3.7*.3*.5 kg  sp_heat=876 J/kg/K  mass_min=1e-6 kg  num_ports=foundation.enum.numPorts2.one  m_specify=off  m_priority=High  m=1 kg  m_nominal_specify=off  m_nominal_value=1  m_nominal_unit=kg  T_specify=on  T_priority=High  T=Ti degC  T_nominal_specify=off  T_nominal_value=1  T_nominal_unit=K  Q_specify=off  Q_priority=None  Q=0 W  Q_nominal_specify=off  Q_nominal_value=1  Q_nominal_unit=W
  Thermal Mass 10-11 : fl_lib/Thermal/Thermal Elements/Thermal Mass  mass_type=foundation.enum.constant_variable.constant  mass=547*.5*.3*12.5 kg  sp_heat=876 J/kg/K  mass_min=1e-6 kg  num_ports=foundation.enum.numPorts2.one  m_specify=off  m_priority=High  m=1 kg  m_nominal_specify=off  m_nominal_value=1  m_nominal_unit=kg  T_specify=on  T_priority=High  T=Ti degC  T_nominal_specify=off  T_nominal_value=1  T_nominal_unit=K  Q_specify=off  Q_priority=None  Q=0 W  Q_nominal_specify=off  Q_nominal_value=1  Q_nominal_unit=W
  Thermal Mass 10-7 : fl_lib/Thermal/Thermal Elements/Thermal Mass  mass_type=foundation.enum.constant_variable.constant  mass=547*1.8*.3*.5 kg  sp_heat=876 J/kg/K  mass_min=1e-6 kg  num_ports=foundation.enum.numPorts2.one  m_specify=off  m_priority=High  m=1 kg  m_nominal_specify=off  m_nominal_value=1  m_nominal_unit=kg  T_specify=on  T_priority=High  T=Ti degC  T_nominal_specify=off  T_nominal_value=1  T_nominal_unit=K  Q_specify=off  Q_priority=None  Q=0 W  Q_nominal_specify=off  Q_nominal_value=1  Q_nominal_unit=W
  Thermal Mass 10-9 : fl_lib/Thermal/Thermal Elements/Thermal Mass  mass_type=foundation.enum.constant_variable.constant  mass=547*.5*.3*12.5 kg  sp_heat=876 J/kg/K  mass_min=1e-6 kg  num_ports=foundation.enum.numPorts2.one  m_specify=off  m_priority=High  m=1 kg  m_nominal_specify=off  m_nominal_value=1  m_nominal_unit=kg  T_specify=on  T_priority=High  T=Ti degC  T_nominal_specify=off  T_nominal_value=1  T_nominal_unit=K  Q_specify=off  Q_priority=None  Q=0 W  Q_nominal_specify=off  Q_nominal_value=1  Q_nominal_unit=W
  Thermal Mass Air : fl_lib/Thermal/Thermal Elements/Thermal Mass  mass_type=foundation.enum.constant_variable.constant  mass=30.3 kg  sp_heat=1005 J/kg/K  mass_min=1e-6 kg  num_ports=foundation.enum.numPorts2.one  m_specify=off  m_priority=High  m=1 kg  m_nominal_specify=off  m_nominal_value=1  m_nominal_unit=kg  T_specify=on  T_priority=High  T=Ti degC  T_nominal_specify=off  T_nominal_value=1  T_nominal_unit=K  Q_specify=off  Q_priority=None  Q=0 W  Q_nominal_specify=off  Q_nominal_value=1  Q_nominal_unit=W
  Thermal Mass Flur10EG : fl_lib/Thermal/Thermal Elements/Thermal Mass  mass_type=foundation.enum.constant_variable.constant  mass=4090 kg  sp_heat=889 J/kg/K  mass_min=1e-6 kg  num_ports=foundation.enum.numPorts2.one  m_specify=off  m_priority=High  m=1 kg  m_nominal_specify=off  m_nominal_value=1  m_nominal_unit=kg  T_specify=on  T_priority=High  T=Ti degC  T_nominal_specify=off  T_nominal_value=1  T_nominal_unit=K  Q_specify=off  Q_priority=None  Q=0 W  Q_nominal_specify=off  Q_nominal_value=1  Q_nominal_unit=W
  Thermal Mass Flur10OG2 : fl_lib/Thermal/Thermal Elements/Thermal Mass  mass_type=foundation.enum.constant_variable.constant  mass=4090 kg  sp_heat=889 J/kg/K  mass_min=1e-6 kg  num_ports=foundation.enum.numPorts2.one  m_specify=off  m_priority=High  m=1 kg  m_nominal_specify=off  m_nominal_value=1  m_nominal_unit=kg  T_specify=on  T_priority=High  T=Ti degC  T_nominal_specify=off  T_nominal_value=1  T_nominal_unit=K  Q_specify=off  Q_priority=None  Q=0 W  Q_nominal_specify=off  Q_nominal_value=1  Q_nominal_unit=W
  Thermal Mass InnerDoor : fl_lib/Thermal/Thermal Elements/Thermal Mass  mass_type=foundation.enum.constant_variable.constant  mass=1.8*.022*450 kg  sp_heat=1600 J/kg/K  mass_min=1e-6 kg  num_ports=foundation.enum.numPorts2.one  m_specify=off  m_priority=High  m=1 kg  m_nominal_specify=off  m_nominal_value=1  m_nominal_unit=kg  T_specify=on  T_priority=High  T=Ti degC  T_nominal_specify=off  T_nominal_value=1  T_nominal_unit=K  Q_specify=off  Q_priority=None  Q=0 W  Q_nominal_specify=off  Q_nominal_value=1  Q_nominal_unit=W
  Thermal Reference1 : fl_lib/Thermal/Thermal Elements/Thermal Reference
  X-Atm : Subsystem
  10-11 : PMIOPort  Side=Left
  Hot Water Out1 : PMIOPort  Port=2  Side=Left
  10-1 : PMIOPort  Port=3  Side=Left
  Hot Water In1 : PMIOPort  Port=4  Side=Left
  10-9 : PMIOPort  Port=5  Side=Right
  Door10 : PMIOPort  Port=6  Side=Right
  10-7 : PMIOPort  Port=7  Side=Right
  Y-Flur10OG2 : PMIOPort  Port=8  Side=Left
  Y-Flur1EG : PMIOPort  Port=9  Side=Left
  Troom : Outport
  wires:
  Temp. Sensor/1(T) -> Troom/1
  Tatm/1 -> Simulink-PS Converter3/1
  valve command/1 -> Heater/1(valve command)
  connections:
  Flur10OG2/RConn1 -- Half Flur10OG2/LConn1
  Half Flur10OG2/RConn1 -- Y-Flur10OG2/RConn1 -- Thermal Mass Flur10OG2/LConn1
  IW10-11/RConn1 -- Half Wall-Air Conduction3/LConn1
  IW10-1/RConn1 -- Half Wall-Air Conduction1/LConn1
  Air-InnerDoor Convection1/RConn1 -- Half Window-Air Conduction1/LConn1
  IW10-7/RConn1 -- Half Wall-Air Conduction2/LConn1
  IW10-9/RConn1 -- Half Wall-Air Conduction4/LConn1
  Thermal Mass 10-7/LConn1 -- Half Wall-Air Conduction2/RConn1 -- 10-7/RConn1
  10-1/RConn1 -- Half Wall-Air Conduction1/RConn1 -- Thermal Mass 10-1/LConn1
  Thermal Mass 10-9/LConn1 -- Half Wall-Air Conduction4/RConn1 -- 10-9/RConn1
  Half Wall-Air Conduction3/RConn1 -- Thermal Mass 10-11/LConn1 -- 10-11/RConn1
  Thermal Mass InnerDoor/LConn1 -- Door10/RConn1 -- Half Window-Air Conduction1/RConn1
  Flur10OG2/LConn1 -- Flur10EG/LConn1 -- Heater/RConn1 -- Thermal Mass Air/LConn1 -- Temp. Sensor/LConn1 -- X-Atm/LConn1 -- Air-InnerDoor Convection1/LConn1 -- IW10-1/LConn1 -- IW10-7/LConn1 -- IW10-9/LConn1 -- IW10-11/LConn1
  Thermal Reference1/LConn1 -- Controlled Temperature Source/RConn2
  Controlled Temperature Source/RConn1 -- Simulink-PS Converter3/RConn1
  X-Atm/RConn1 -- Controlled Temperature Source/LConn1
  Hot Water In1/RConn1 -- Heater/LConn1
  Heater/RConn2 -- Hot Water Out1/RConn1
  Half Flur10EG/RConn1 -- Thermal Mass Flur10EG/LConn1 -- Y-Flur1EG/RConn1
  Flur10EG/RConn1 -- Half Flur10EG/LConn1
